simulink model "main_simulation"  (R2026b)
settings: Solver=ode4  StopTime=60.0  FixedStep=0.01
settings Model: Creator=MSI1  LastModifiedBy=MSI1

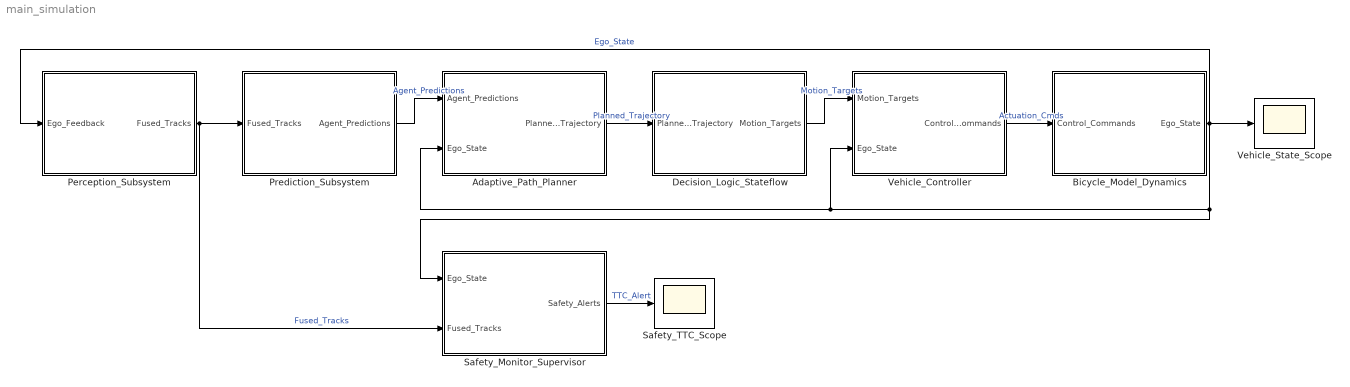
== system main_simulation ==
  Adaptive_Path_Planner : Subsystem
  Bicycle_Model_Dynamics : Subsystem
  Decision_Logic_Stateflow : Subsystem
  Perception_Subsystem : Subsystem
  Prediction_Subsystem : Subsystem
  Safety_Monitor_Supervisor : Subsystem
  Safety_TTC_Scope : Scope
  Vehicle_Controller : Subsystem
  Vehicle_State_Scope : Scope
  wires:
  Perception_Subsystem/1(Fused_Tracks) -> Prediction_Subsystem/1(Fused_Tracks), Safety_Monitor_Supervisor/2(Fused_Tracks)  "Fused_Tracks"
  Prediction_Subsystem/1(Agent_Predictions) -> Adaptive_Path_Planner/1(Agent_Predictions)  "Agent_Predictions"
  Adaptive_Path_Planner/1(Planned_Trajectory) -> Decision_Logic_Stateflow/1(Planned_Trajectory)  "Planned_Trajectory"
  Decision_Logic_Stateflow/1(Motion_Targets) -> Vehicle_Controller/1(Motion_Targets)  "Motion_Targets"
  Vehicle_Controller/1(Control_Commands) -> Bicycle_Model_Dynamics/1(Control_Commands)  "Actuation_Cmds"
  Bicycle_Model_Dynamics/1(Ego_State) -> Adaptive_Path_Planner/2(Ego_State), Vehicle_Controller/2(Ego_State), Safety_Monitor_Supervisor/1(Ego_State), Vehicle_State_Scope/1, Perception_Subsystem/1(Ego_Feedback)  "Ego_State"
  Safety_Monitor_Supervisor/1(Safety_Alerts) -> Safety_TTC_Scope/1  "TTC_Alert"

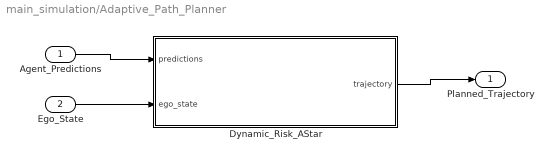
== system main_simulation/Adaptive_Path_Planner ==
  Agent_Predictions : Inport
  Ego_State : Inport  Port=2
  Dynamic_Risk_AStar : MATLAB Function  TreatAsAtomicUnit=on
  Planned_Trajectory : Outport
  wires:
  Agent_Predictions/1 -> Dynamic_Risk_AStar/1(predictions)
  Ego_State/1 -> Dynamic_Risk_AStar/2(ego_state)
  Dynamic_Risk_AStar/1(trajectory) -> Planned_Trajectory/1

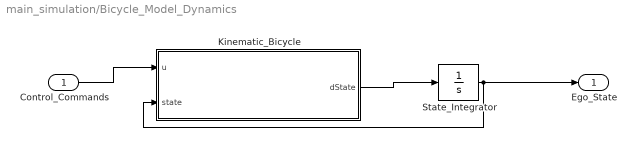
== system main_simulation/Bicycle_Model_Dynamics ==
  Control_Commands : Inport
  Kinematic_Bicycle : MATLAB Function  TreatAsAtomicUnit=on
  State_Integrator : Integrator  InitialCondition=[0; 1.5; 8.0; 0]
  Ego_State : Outport
  wires:
  Control_Commands/1 -> Kinematic_Bicycle/1(u)
  Kinematic_Bicycle/1(dState) -> State_Integrator/1
  State_Integrator/1 -> Ego_State/1, Kinematic_Bicycle/2(state)

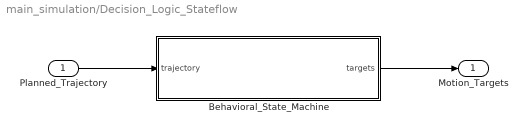
== system main_simulation/Decision_Logic_Stateflow ==
  Planned_Trajectory : Inport
  Behavioral_State_Machine : MATLAB Function  TreatAsAtomicUnit=on
  Motion_Targets : Outport
  wires:
  Planned_Trajectory/1 -> Behavioral_State_Machine/1(trajectory)
  Behavioral_State_Machine/1(targets) -> Motion_Targets/1

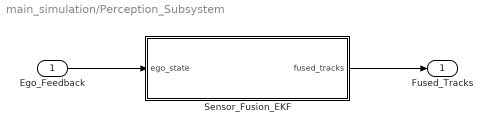
== system main_simulation/Perception_Subsystem ==
  Ego_Feedback : Inport
  Sensor_Fusion_EKF : MATLAB Function  TreatAsAtomicUnit=on
  Fused_Tracks : Outport
  wires:
  Ego_Feedback/1 -> Sensor_Fusion_EKF/1(ego_state)
  Sensor_Fusion_EKF/1(fused_tracks) -> Fused_Tracks/1

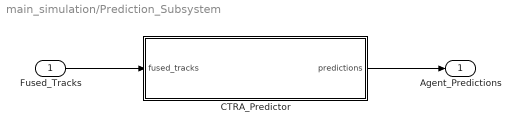
== system main_simulation/Prediction_Subsystem ==
  Fused_Tracks : Inport
  CTRA_Predictor : MATLAB Function  TreatAsAtomicUnit=on
  Agent_Predictions : Outport
  wires:
  Fused_Tracks/1 -> CTRA_Predictor/1(fused_tracks)
  CTRA_Predictor/1(predictions) -> Agent_Predictions/1

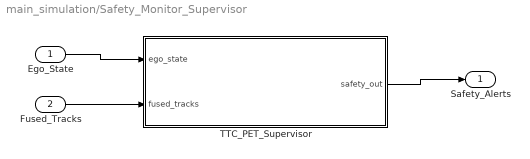
== system main_simulation/Safety_Monitor_Supervisor ==
  Ego_State : Inport
  Fused_Tracks : Inport  Port=2
  TTC_PET_Supervisor : MATLAB Function  TreatAsAtomicUnit=on
  Safety_Alerts : Outport
  wires:
  Ego_State/1 -> TTC_PET_Supervisor/1(ego_state)
  Fused_Tracks/1 -> TTC_PET_Supervisor/2(fused_tracks)
  TTC_PET_Supervisor/1(safety_out) -> Safety_Alerts/1

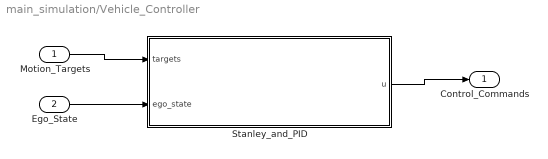
== system main_simulation/Vehicle_Controller ==
  Motion_Targets : Inport
  Ego_State : Inport  Port=2
  Stanley_and_PID : MATLAB Function  TreatAsAtomicUnit=on
  Control_Commands : Outport
  wires:
  Motion_Targets/1 -> Stanley_and_PID/1(targets)
  Ego_State/1 -> Stanley_and_PID/2(ego_state)
  Stanley_and_PID/1(u) -> Control_Commands/1

== matlab function main_simulation/Perception_Subsystem/Sensor_Fusion_EKF ==
  data: ego_state input; fused_tracks output
function fused_tracks = Sensor_Fusion_EKF(ego_state)
% Multi-Sensor Fusion & Road Surface Estimator
% Fuses Camera (120m), LiDAR (80m), Radar (110m)
fused_tracks = zeros(10, 6);
fused_tracks(1, :) = [1, 2, 85, 1.5, -10, 0]; % Oncoming Truck
fused_tracks(2, :) = [2, 5, 20, 2.2, 3, 0];   % Bicycle
fused_tracks(3, :) = [3, 7, 75, 4.0, 0, -1];  % Crossing Cattle
end

== matlab function main_simulation/Adaptive_Path_Planner/Dynamic_Risk_AStar ==
  data: predictions input; trajectory output; ego_state input
function trajectory = Dynamic_Risk_AStar(predictions, ego_state)
% Dynamic Risk Grid & Spatiotemporal Frenet Path Planner
trajectory = zeros(50, 4);
for k = 1:50
    s = (k - 1) * 1.5;
    trajectory(k, 1) = ego_state(1) + s * cos(ego_state(4));
    trajectory(k, 2) = ego_state(2) + s * sin(ego_state(4));
    trajectory(k, 3) = 8.0;
    trajectory(k, 4) = 0.0;
end
end

== matlab function main_simulation/Decision_Logic_Stateflow/Behavioral_State_Machine ==
  data: trajectory input; targets output
function targets = Behavioral_State_Machine(trajectory)
% State Arbitration: Cruise | Yield | Overtake | Stop
targets = [trajectory(10, 1), trajectory(10, 2), trajectory(10, 3), 0.0];
end

== matlab function main_simulation/Vehicle_Controller/Stanley_and_PID ==
  data: targets input; u output; ego_state input
function u = Stanley_and_PID(targets, ego_state)
% Stanley Lateral Steering + Longitudinal Speed PID Controller
e_fa = -(ego_state(1) - targets(1)) * sin(ego_state(4)) + (ego_state(2) - targets(2)) * cos(ego_state(4));
delta = (0 - ego_state(4)) + atan2(0.5 * e_fa, max(ego_state(3), 1.0));
delta = max(min(delta, 0.6), -0.6);
a_x = max(min(1.2 * (targets(3) - ego_state(3)), 3.0), -6.0);
u = [delta; a_x];
end

== matlab function main_simulation/Bicycle_Model_Dynamics/Kinematic_Bicycle ==
  data: u input; dState output; state input
function dState = Kinematic_Bicycle(u, state)
% Nonlinear Kinematic Bicycle Equations of Motion
L = 2.8; lr = 1.4;
beta = atan(lr / L * tan(u(1)));
x_dot = state(3) * cos(state(4) + beta);
y_dot = state(3) * sin(state(4) + beta);
v_dot = u(2);
psi_dot = (state(3) / lr) * sin(beta);
dState = [x_dot; y_dot; v_dot; psi_dot];
end

== matlab function main_simulation/Safety_Monitor_Supervisor/TTC_PET_Supervisor ==
  data: ego_state input; safety_out output; fused_tracks input
function safety_out = TTC_PET_Supervisor(ego_state, fused_tracks)
% Deterministic Time-To-Collision (TTC) & PET Supervisor
min_ttc = 99.0; aeb_trigger = 0.0;
for i = 1:size(fused_tracks, 1)
    if fused_tracks(i, 1) > 0
        dx = fused_tracks(i, 3) - ego_state(1);
        dv = ego_state(3) - fused_tracks(i, 5);
        if dx > 0 && dv > 0.1
            ttc = dx / dv;
            if ttc < min_ttc, min_ttc = ttc; end
        end
    end
end
if min_ttc < 1.5, aeb_trigger = 1.0; end
safety_out = [min_ttc; aeb_trigger];
end

== matlab function main_simulation/Prediction_Subsystem/CTRA_Predictor ==
  data: fused_tracks input; predictions output
function predictions = CTRA_Predictor(fused_tracks)
% Heterogeneous CTRA multi-modal trajectory prediction
predictions = zeros(10, 30, 3);
for i = 1:size(fused_tracks, 1)
    if fused_tracks(i, 1) > 0
        for t = 1:30
            predictions(i, t, 1) = fused_tracks(i, 3) + fused_tracks(i, 5) * (t * 0.1);
            predictions(i, t, 2) = fused_tracks(i, 4) + fused_tracks(i, 6) * (t * 0.1);
            predictions(i, t, 3) = 0.8;
        end
    end
end
end
